simulink model "Vejlupek_CAR4_dsPIC33_ACU44_SPI_R02"  (Simulink 7.3)
settings: Solver=FixedStepDiscrete  StartTime=0.0  StopTime=10.0  FixedStep=0.01  RelTol=1e-3
undefined symbols (not defined in the file or in its folder): PWM, QEIInit
libraries: dsPICdrivers x19, simulink x2
settings Model: Creator=Lubin  LastModifiedBy=Bobes
settings OptimizationCC: InlineParams=on  InlineInvariantSignals=on  InitFltsAndDblsToZero=on  OptimizeModelRefInitCode=on  LifeSpan=1
settings DebuggingCC: SaveWithParameterizedLinksMsg=none  SignalResolutionControl=TryResolveAllWithWarning
settings HardwareCC: ProdBitPerInt=16  ProdEndianess=LittleEndian  ProdWordSize=16  ProdHWDeviceType=16-bit Generic  TargetHWDeviceType=32-bit Generic
settings RTWCC: SystemTargetFile=dspic.tlc  TemplateMakefile=dspic_pic30_gcc.tmf  PostCodeGenCommand=dsPIC_Compile()  Description=Embedded Target for Microchip dsPIC (real-time)  GenerateReport=on  ProcessScript=dspic_make_rtw_hook  CustomSource=QEI_Functions.c  IncludeHyperlinkInReport=on  LaunchReport=on  GenerateTraceInfo=on  GenerateTraceReport=on  GenerateTraceReportSl=on  GenerateTraceReportSf=on  GenerateTraceReportEml=on
settings CodeAppCC: IgnoreCustomStorageClasses=off
settings STFCustomTargetCC: ModelReferenceCompliant=off  IncludeMdlTerminateFcn=off  CombineOutputUpdateFcns=on  SuppressErrorStatus=on  ERTCustomFileBanners=on  SupportContinuousTime=off  SupportNonInlinedSFcns=off  SystemTargetFile=dspic.tlc
settings ERTTargetCC: MultiwordLength=2048  ModelReferenceCompliant=off  ParMdlRefBuildCompliant=off  CompOptLevelCompliant=off  IncludeMdlTerminateFcn=off  SuppressErrorStatus=on  ERTFirstTimeCompliant=off  ModelStepFunctionPrototypeControlCompliant=off  CPPClassGenCompliant=off  InlinedParameterPlacement=NonHierarchical  ERTSrcFileBannerTemplate=dsPIC_code_template.cgt  ERTHdrFileBannerTemplate=dsPIC_code_template.cgt  ERTDataSrcFileTemplate=dsPIC_code_template.cgt  ERTDataHdrFileTemplate=dsPIC_code_template.cgt  ERTCustomFileTemplate=dsPIC_main.tlc
settings CustomProperty: DataType=string  Value=C:\PROGRA~1\MATLAB\R2009a\bin\win32\gmake

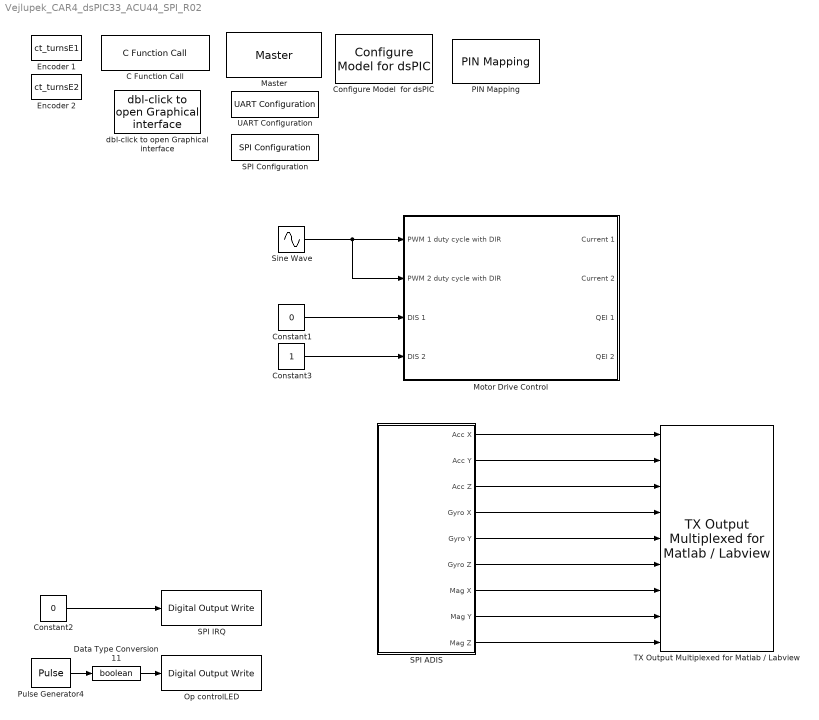
== system Vejlupek_CAR4_dsPIC33_ACU44_SPI_R02 ==
  C Function Call : dsPICdrivers/OTHERS/C Function Call  Tag=dsPIC_dsPIC_CFunctionCall  fctName='QEIInit'  INPUT_SIZE=1  INPUT1=--  INPUT2=--  INPUT3=--  OUTPUT_SIZE=1  OUTPUT1=--  SampleTime=inf  InputType=[ ]  OutputType=[ ]  FctDeclaration=extern void QEIInit();  FctCall=QEIInit();  OrderingInOutPopup=None
  Configure Model  for dsPIC : dsPICdrivers/Simulink Configuration/Configure Model  for dsPIC
  Constant1 : Constant  Value=0  OutDataTypeMode=boolean  OutDataType=fixdt(1, 16)  OutScaling=2^0  OutDataTypeStr=boolean  SampleTime=0.01
  Constant2 : Constant  Value=0  OutDataTypeMode=boolean  OutDataType=fixdt(1, 16)  OutScaling=2^0  OutDataTypeStr=boolean  SampleTime=0.01
  Constant3 : Constant  OutDataTypeMode=boolean  OutDataType=fixdt(1, 16)  OutScaling=2^0  OutDataTypeStr=boolean  SampleTime=0.01
  Data Type Conversion11 : DataTypeConversion  OutDataTypeMode=boolean  OutDataType=fixdt(1, 16)  OutScaling=2^0  OutDataTypeStr=boolean
  Encoder 1 : DataStoreMemory  DataStoreName=ct_turnsE1  ReadBeforeWriteMsg=warning  WriteAfterWriteMsg=warning  WriteAfterReadMsg=warning  DataType=uint16  OutDataType=sfix(16)  OutScaling=2^0  OutDataTypeStr=uint16
      settings: RTWStateStorageClass=ExportedGlobal
  Encoder 2 : DataStoreMemory  DataStoreName=ct_turnsE2  ReadBeforeWriteMsg=warning  WriteAfterWriteMsg=warning  WriteAfterReadMsg=warning  DataType=uint16  OutDataType=sfix(16)  OutScaling=2^0  OutDataTypeStr=uint16
      settings: RTWStateStorageClass=ExportedGlobal
  Master : dsPICdrivers/Master  Tag=dsPIC_MASTER  Priority=1  TimeStepType=Timer1  picType=33fj128MC804  fcy=20000000  Quartz_33f=20e6  PLLActive_33f=on  fcyDesired_33f=20000000  tmr1="[8  24999  0]"  tmr1Info="Time Step : 0.01  ;   Error : 0%  PR1=24999"  tmr2345="[0  0  0  0]"  tmr2345cfg=[-1 -1 -1 -1]  IOautoConf=on  typePort="[ 8   8   0   0   0   0   0  10  10   0  10   0   0   0   0   0   0   0  22  22  23   0   0  23  22  21  10   0   0   0   0   0  22  22  22  23   0   0  10   0   0  10   0   0   0   0   0   0   0   0   0   0   0   0   0   0   0   0   0   0   0   0   0   0   0   0   0   0   0   0   0   0   0   0   0   0   0   0   0   0   0   0   0   0   0   0   0   0   0   0   0   0   0   0   0   0   0   0   0   0   0   0   0   0   0   0   0   0   0   0   0   0 ]"  TRIS="[ 64127  63855  64951  65535  65535  65535  65535 ]"  ADPCFG=496  MasterBusyPort=None  MasterOverloadPort=None  FOSC=Quartz (XT - HS)  ClockSwitchMonitor=Both disabled  TempProtection_33f=TEMP_ON  FPBOR=<empty>  PWRT=64ms  MCLR=<empty>  PowerSave=off  OverrideFcy=off  NewFcy=1e6  PR2345="[65535  65535  65535  65535]"
  Motor Drive Control : Subsystem
  Op controlLED : dsPICdrivers/Digital I//O/Digital Output Write  Tag=dsPIC_Digital_Output  Priority=5  PORT=A  Pin=[8]  Simultaneous=off  OrderingInOutPopup=None
  PIN Mapping : dsPICdrivers/Peripheral MAPPING/PIN Mapping  Tag=dsPIC_PIN_Mapping  in_INT1=Not tied (VSS)  in_INT2=Not tied (VSS)  in_T2CK=Not tied (VSS)  in_T3CK=Not tied (VSS)  in_T4CK=Not tied (VSS)  in_T5CK=Not tied (VSS)  in_IC1=Not tied (VSS)  in_IC2=Not tied (VSS)  in_IC7=Not tied (VSS)  in_IC8=Not tied (VSS)  out_OC1=Not changed  out_OC2=Not changed  out_OC3=Not changed  out_OC4=Not changed  in_OCFA=Not tied (VSS)  in_FLTA1=Not tied (VSS)  in_FLTA2=Not tied (VSS)  in_QEA1=tied to RP16  in_QEB1=tied to RP17  in_INDX1=Not tied (VSS)  out_UPDN1=Not changed  out_UPDN2=Not changed  in_QEA2=tied to RP2  in_QEB2=tied to RP3  in_INDX2=Not tied (VSS)  in_U1RX=tied to RP18  out_U1TX=tied to RP4  in_U1CTS=Not tied (VSS)  out_U1RTS=Not changed  in_U2RX=Not changed  out_U2TX=Not changed  in_U2CTS=Not tied (VSS)  out_U2RTS=Not changed  in_SDI1=tied to RP8  out_SDO1=tied to RP19  in_SCK1=Not tied (VSS)  out_SCK1OUT=tied to RP7  in_SS1=Not tied (VSS)  out_SS1OUT=Not changed  in_SDI2=Not tied (VSS)  out_SDO2=Not changed  in_SCK2=Not tied (VSS)  out_SCK2OUT=Not changed  in_SS2=Not tied (VSS)  out_SS2OUT=Not changed  in_C1RX=Not tied (VSS)  out_C1TX=Not changed  out_C1OUT=Not changed  out_C2OUT=Not changed
  Pulse Generator4 : DiscretePulseGenerator  Amplitude=1  Period=100  PulseWidth=50  PhaseDelay=0  SampleTime=0.01
  SPI ADIS : Subsystem
  SPI Configuration : dsPICdrivers/SPI PORT/SPI Configuration  Tag=dsPIC_config_SPI  Priority=2  ConfigurationTime=At boot time (only once)  OrderingInOutPopup=None  SampleTime=-1  Frame_Enable=0  Frame_Sync=None  SPI=1  MODE=MASTER  USER_SCALER=96  StartEnable=Enable  SDO_EN=on  DATA_LENGTH=16 bits  SS_EN=off  SMP=Middle of bit  CKP=high  CKE=Idle to Active  Status="OK - Mode 1  -    Fsck= 208333.3333Hz"
  SPI IRQ : dsPICdrivers/Digital I//O/Digital Output Write  Tag=dsPIC_Digital_Output  Priority=5  PORT=C  Pin=[6]  Simultaneous=off  OrderingInOutPopup=None
  Sine Wave : Sin  SineType=Sample based  Amplitude=PWM*0.9  Bias=0  Frequency=1  Phase=0  Samples=10e2  SampleTime=1e-2  Offset=0
  TX Output Multiplexed for Matlab / Labview : dsPICdrivers/Serial PORT/TX Output Multiplexed for Matlab // Labview  Tag=dsPIC_TX_Multiplexed  Priority=5  UART=1  CleverSpreadingChk=on  CleverSpreading=1  CHANNEL=[0 1 2 3 4 5 6 7 8]  CHANNELBLOCKED=[]  CHANNELBLOCKED_BITEWISE=0  Status=OK
  UART Configuration : dsPICdrivers/Serial PORT/UART Configuration  Tag=dsPIC_config_UART  Priority=2  UART=1  proposed_BAUD=9600  ALT_TX_RX=on  InterruptTxWhen=When Transmit Buffer is empty  TXInterruptPri=1  TxBufferSize=32  TXEN=on  InterruptRxWhen=When Receive Buffer is full (contain 4 characters)  RXInterruptPri=2  RxBufferSize=32  BAUD=9600  UxBRG=129  Info="UxBRG = 129   ||  Real Baud : 9615   ||  % error : 0.16026  ||  max 9.6154 Bytes / Step"  RealBaud=0
  dbl-click to open Graphical interface : dsPICdrivers/Serial PORT/dbl-click to open Graphical interface  SystemSampleTime=-1  Nothing=0
  wires:
  Sine Wave/1 -> Motor Drive Control/1(PWM 1 duty cycle with DIR), Motor Drive Control/2(PWM 2 duty cycle with DIR)
  Data Type Conversion11/1 -> Op controlLED/1
  Pulse Generator4/1 -> Data Type Conversion11/1
  Constant1/1 -> Motor Drive Control/3(DIS 1)
  Constant3/1 -> Motor Drive Control/4(DIS 2)
  Constant2/1 -> SPI IRQ/1
  SPI ADIS/1(Acc X) -> TX Output Multiplexed for Matlab / Labview/1
  SPI ADIS/2(Acc Y) -> TX Output Multiplexed for Matlab / Labview/2
  SPI ADIS/3(Acc Z) -> TX Output Multiplexed for Matlab / Labview/3
  SPI ADIS/4(Gyro X) -> TX Output Multiplexed for Matlab / Labview/4
  SPI ADIS/5(Gyro Y) -> TX Output Multiplexed for Matlab / Labview/5
  SPI ADIS/6(Gyro Z) -> TX Output Multiplexed for Matlab / Labview/6
  SPI ADIS/7(Mag X) -> TX Output Multiplexed for Matlab / Labview/7
  SPI ADIS/8(Mag Y) -> TX Output Multiplexed for Matlab / Labview/8
  SPI ADIS/9(Mag Z) -> TX Output Multiplexed for Matlab / Labview/9

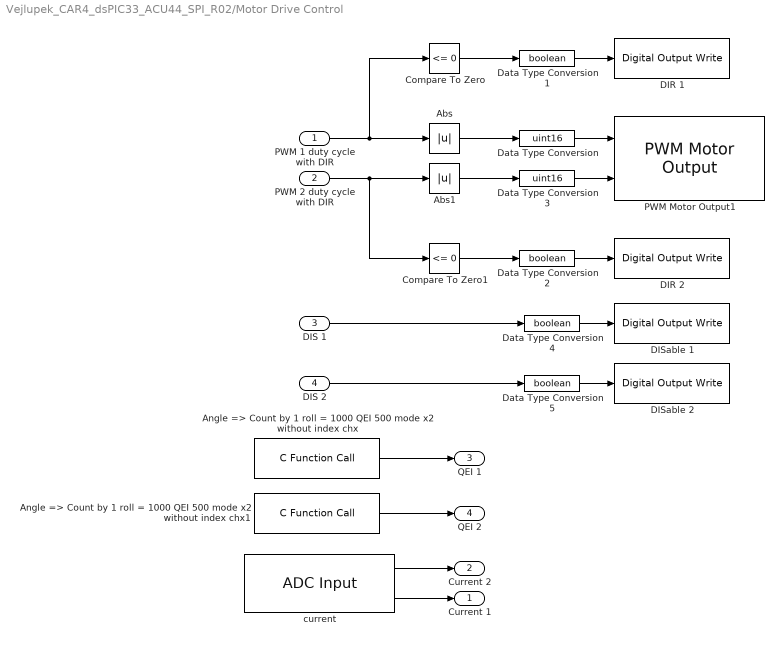
== system Vejlupek_CAR4_dsPIC33_ACU44_SPI_R02/Motor Drive Control ==
  PWM 1 duty cycle with DIR : Inport
  PWM 2 duty cycle with DIR : Inport  Port=2
  DIS 1 : Inport  Port=3
  DIS 2 : Inport  Port=4
  Abs : Abs  OutDataType=fixdt(1, 16)  OutScaling=2^0
  Abs1 : Abs  OutDataType=fixdt(1, 16)  OutScaling=2^0
  Angle => Count by 1 roll = 1000 QEI 500 mode x2 without index chx : dsPICdrivers/OTHERS/C Function Call  Tag=dsPIC_dsPIC_CFunctionCall  fctName='GetQEI1'  INPUT_SIZE=1  INPUT1=--  INPUT2=--  INPUT3=--  OUTPUT_SIZE=1  OUTPUT1=uint16  SampleTime=-1  InputType=[ ]  OutputType=[ 4 ]  FctDeclaration=extern uint16_T GetQEI1();  FctCall=%y1 = GetQEI1();  OrderingInOutPopup=None
  Angle => Count by 1 roll = 1000 QEI 500 mode x2 without index chx1 : dsPICdrivers/OTHERS/C Function Call  Tag=dsPIC_dsPIC_CFunctionCall  fctName='GetQEI2'  INPUT_SIZE=1  INPUT1=--  INPUT2=--  INPUT3=--  OUTPUT_SIZE=1  OUTPUT1=uint16  SampleTime=-1  InputType=[ ]  OutputType=[ 4 ]  FctDeclaration=extern uint16_T GetQEI2();  FctCall=%y1 = GetQEI2();  OrderingInOutPopup=None
  Compare To Zero : simulink/Logic and Bit Operations/Compare To Zero  SystemSampleTime=-1  relop=<=  LogicOutDataTypeMode=boolean  ZeroCross=off
  Compare To Zero1 : simulink/Logic and Bit Operations/Compare To Zero  SystemSampleTime=-1  relop=<=  LogicOutDataTypeMode=boolean  ZeroCross=off
  DIR 1 : dsPICdrivers/Digital I//O/Digital Output Write  Tag=dsPIC_Digital_Output  Priority=5  PORT=A  Pin=[10]  Simultaneous=off  OrderingInOutPopup=None
  DIR 2 : dsPICdrivers/Digital I//O/Digital Output Write  Tag=dsPIC_Digital_Output  Priority=5  PORT=B  Pin=[10]  Simultaneous=off  OrderingInOutPopup=None
  DISable 1 : dsPICdrivers/Digital I//O/Digital Output Write  Tag=dsPIC_Digital_Output  Priority=5  PORT=A  Pin=[7]  Simultaneous=off  OrderingInOutPopup=None
  DISable 2 : dsPICdrivers/Digital I//O/Digital Output Write  Tag=dsPIC_Digital_Output  Priority=5  PORT=C  Pin=[9]  Simultaneous=off  OrderingInOutPopup=None
  Data Type Conversion : DataTypeConversion  OutDataTypeMode=uint16  OutDataType=fixdt(1, 16)  OutScaling=2^0  OutDataTypeStr=uint16
  Data Type Conversion{1..2,4..5} (4 alike) : DataTypeConversion  OutDataTypeMode=boolean  OutDataType=fixdt(1, 16)  OutScaling=2^0  OutDataTypeStr=boolean
  Data Type Conversion3 : DataTypeConversion  OutDataTypeMode=uint16  OutDataType=fixdt(1, 16)  OutScaling=2^0  OutDataTypeStr=uint16
  PWM Motor Output1 : dsPICdrivers/Peripheral I//O/PWM Motor Output  Tag=dsPIC_PWM_Motor  Priority=5  PWMref=1  PWM12=2  InputEnableChk=off  InputPeriodeChk=off  Channel=[1 2]  TPeriode=.0001  PrescalerValue=1  PeriodeInteger=2000  MaxName='PWM'  Centered=off  HChannelON=off  Info="Nbr Bits : 11.9658  ||  PWM = 4000  ||  Prescaler = 1"  Delay=0  IntPriority=5  nbrPwmChannelPIC=3  Status=OK  DeadTimePrescaleA=0  DeadTimePrescaleB=0  DeadTimeInfo="Dead Time A = 0  ||  Dead Time B = 0"  DTPWM1a=Prescaler A  DTPWM1i=Prescaler A  DTPWM2a=Prescaler A  DTPWM2i=Prescaler A  DTPWM3a=Prescaler A  DTPWM3i=Prescaler A  DTPWM4a=Prescaler A  DTPWM4i=Prescaler A  DTCON1=0  DTCON2=0
  current : dsPICdrivers/Peripheral I//O/ADC Input  Tag=dsPIC_ADC  Priority=5  ADC_TYPE=12 bits  ADC_MODE=Continuous sampling & get last channel value  NbrSampleStep=1  VoltRefpopup="AVdd  -  AVss"  OutFormatBitspopup=0000 dddd dddd dddd : Integer  InterruptPriority=6  ANCHANNELS=[0 1]  MaxName=ANmax = 4095  Rin=1e2  ADCS=26  SAMC=1  Temperature=25  DMAChannel=0  SampleTime=0.01  Status="OK  |  Tsmp=6.750e-007 |  T/Channel=1.012e-005 |  Tall=2.025e-005"  SSRC=auto convert
  Current 1 : Outport
  Current 2 : Outport  Port=2
  QEI 1 : Outport  Port=3
  QEI 2 : Outport  Port=4
  wires:
  Data Type Conversion1/1 -> DIR 1/1
  Data Type Conversion/1 -> PWM Motor Output1/1
  Compare To Zero/1 -> Data Type Conversion1/1
  PWM 1 duty cycle with DIR/1 -> Compare To Zero/1, Abs/1
  Abs/1 -> Data Type Conversion/1
  Angle => Count by 1 roll = 1000 QEI 500 mode x2 without index chx1/1 -> QEI 2/1
  Angle => Count by 1 roll = 1000 QEI 500 mode x2 without index chx/1 -> QEI 1/1
  PWM 2 duty cycle with DIR/1 -> Abs1/1, Compare To Zero1/1
  Abs1/1 -> Data Type Conversion3/1
  Compare To Zero1/1 -> Data Type Conversion2/1
  Data Type Conversion2/1 -> DIR 2/1
  Data Type Conversion3/1 -> PWM Motor Output1/2
  DIS 1/1 -> Data Type Conversion4/1
  DIS 2/1 -> Data Type Conversion5/1
  Data Type Conversion4/1 -> DISable 1/1
  Data Type Conversion5/1 -> DISable 2/1
  current/1 -> Current 2/1
  current/2 -> Current 1/1

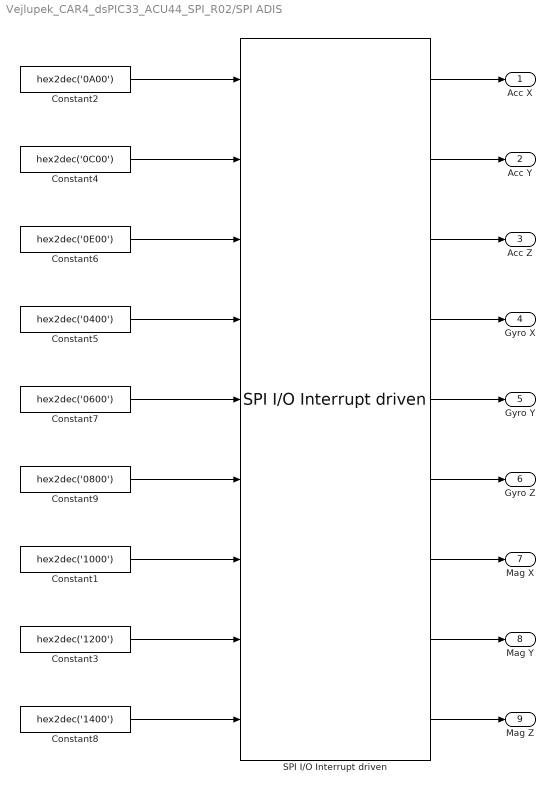
== system Vejlupek_CAR4_dsPIC33_ACU44_SPI_R02/SPI ADIS ==
  Constant1 : Constant  Value=hex2dec('1000')  VectorParams1D=off  OutDataTypeMode=uint16  OutDataType=sfix(16)  OutScaling=2^0  OutDataTypeStr=uint16  SampleTime=-1
  Constant2 : Constant  Value=hex2dec('0A00')  VectorParams1D=off  OutDataTypeMode=uint16  OutDataType=sfix(16)  OutScaling=2^0  OutDataTypeStr=uint16  SampleTime=-1
  Constant3 : Constant  Value=hex2dec('1200')  VectorParams1D=off  OutDataTypeMode=uint16  OutDataType=sfix(16)  OutScaling=2^0  OutDataTypeStr=uint16  SampleTime=-1
  Constant4 : Constant  Value=hex2dec('0C00')  VectorParams1D=off  OutDataTypeMode=uint16  OutDataType=sfix(16)  OutScaling=2^0  OutDataTypeStr=uint16  SampleTime=-1
  Constant5 : Constant  Value=hex2dec('0400')  VectorParams1D=off  OutDataTypeMode=uint16  OutDataType=sfix(16)  OutScaling=2^0  OutDataTypeStr=uint16  SampleTime=-1
  Constant6 : Constant  Value=hex2dec('0E00')  VectorParams1D=off  OutDataTypeMode=uint16  OutDataType=sfix(16)  OutScaling=2^0  OutDataTypeStr=uint16  SampleTime=-1
  Constant7 : Constant  Value=hex2dec('0600')  VectorParams1D=off  OutDataTypeMode=uint16  OutDataType=sfix(16)  OutScaling=2^0  OutDataTypeStr=uint16  SampleTime=-1
  Constant8 : Constant  Value=hex2dec('1400')  VectorParams1D=off  OutDataTypeMode=uint16  OutDataType=sfix(16)  OutScaling=2^0  OutDataTypeStr=uint16  SampleTime=-1
  Constant9 : Constant  Value=hex2dec('0800')  VectorParams1D=off  OutDataTypeMode=uint16  OutDataType=sfix(16)  OutScaling=2^0  OutDataTypeStr=uint16  SampleTime=-1
  SPI I/O Interrupt driven : dsPICdrivers/SPI PORT/SPI I//O Interrupt driven  Tag=dsPIC_SPI_IO_Interrupt  SPI=1  nbrTrame=9  mode=continuous run - Interrupt always enable  Disable=on  DATA_LENGTH=16 bits  OrderingInOutPopup=None  SampleTime=0.01  T1CSL=B9  T1CSH=None  T2CSL=B9  T2CSH=None  T3CSL=B9  T3CSH=None  T4CSL=B9  T4CSH=None  T5CSL=B9  T5CSH=None  T6CSL=B9  T6CSH=None  T7CSL=B9  T7CSH=None  T8CSL=B9  T8CSH=None  T9CSL=B9  T9CSH=None  T10CSL=None  T10CSH=None  T11CSL=None  T11CSH=None  T12CSL=None  T12CSH=None  T13CSL=None  T13CSH=None  T14CSL=None  T14CSH=None  T15CSL=None  T15CSH=None
  Acc X : Outport
  Acc Y : Outport  Port=2
  Acc Z : Outport  Port=3
  Gyro X : Outport  Port=4
  Gyro Y : Outport  Port=5
  Gyro Z : Outport  Port=6
  Mag X : Outport  Port=7
  Mag Y : Outport  Port=8
  Mag Z : Outport  Port=9
  wires:
  SPI I/O Interrupt driven/1 -> Acc X/1
  SPI I/O Interrupt driven/2 -> Acc Y/1
  SPI I/O Interrupt driven/3 -> Acc Z/1
  SPI I/O Interrupt driven/4 -> Gyro X/1
  SPI I/O Interrupt driven/5 -> Gyro Y/1
  SPI I/O Interrupt driven/6 -> Gyro Z/1
  SPI I/O Interrupt driven/7 -> Mag X/1
  SPI I/O Interrupt driven/8 -> Mag Y/1
  SPI I/O Interrupt driven/9 -> Mag Z/1
  Constant5/1 -> SPI I/O Interrupt driven/4
  Constant7/1 -> SPI I/O Interrupt driven/5
  Constant9/1 -> SPI I/O Interrupt driven/6
  Constant1/1 -> SPI I/O Interrupt driven/7
  Constant3/1 -> SPI I/O Interrupt driven/8
  Constant8/1 -> SPI I/O Interrupt driven/9
  Constant2/1 -> SPI I/O Interrupt driven/1
  Constant4/1 -> SPI I/O Interrupt driven/2
  Constant6/1 -> SPI I/O Interrupt driven/3
